simulink model "finalmodel1"  (R2024b)
settings: Solver=FixedStepDiscrete  StartTime=0.0  StopTime=110  FixedStep=SampleTime  MaxStep=1e-3  RelTol=1e-4  AbsTol=1e-3
InitFcn:
  | Ts=50e-6; SampleTime=50e-6; PSSMODEL=1;
  | MB=[1   0.2 30   1.25 40    12 160];
  | 
  | k=[8.3222    2.6014   19.0811    1.9818    3.6841   19.1783  240.6785    2.5684    4.3666   58.7391 7.6960   47.7975    8.7139  296.2463    2.7543    6.5051   47.7755    0.4780   35.4950   18.1866 94.2186]
  | k1=k(1);
  | k2=k(2);
  | k3=k(3);
  | k4=k(4);
  | k5=k(5);
  | k6=k(6);
  | k7=k(7);
  | k8=k(8);
  | k9=k(9);
  | k10=k(10);
  | k11=k(11);
  | k12=k(12);
  | k13=k(13);
  | k14=k(14);
  | k15=k(15);
  | k16=k(16);
  | k17=k(17);
  | k18=k(18);
  | k19=k(19);
  | k20=k(20);
  | k21=k(21);
undefined symbols (not defined in the file or in its folder): dEgdT, DiscIntNeverNeededParam, EgRef, gcbh, Rsh_array5pc, sigbuilder_block, sps_rtmsupport, Tref_K, VT_ref
libraries: spsThreePhaseVIMeasurementLib x14, spsLoadFlowBusLib x9, spsThreePhasePISectionLineLib x6, spsSeriesRLCBranchLib x5, spsThreePhaseTransformerTwoWindingsLib x4, slpidlib x4, spsThreePhaseParallelRLCLoadLib x4, spsThreePhaseSeriesRLCBranchLib x3, spsAlphaBetaZerotodq0Lib x2, spsSynchronousMachinepuStandardLib x2, spsExcitationSystemLib x2, spsMultiBandPowerSystemStabilizerLib x2
(part 1 of 9)
settings Model: Creator=jp536285  LastModifiedBy=Raju
settings SolverCC: AutoScaleAbsTol=off  InitialStep=1e-5  ZeroCrossControl=DisableAll  AlgebraicLoopSolver=TrustRegion  AutoInsertRateTranBlk=on
settings DataIOCC: MaxDataPoints=100000
settings OptimizationCC: LifeSpan=inf
settings DebuggingCC: UnderspecifiedInitializationDetection=Classic  MergeDetectMultiDrivingBlocksExec=none  MultiTaskRateTransMsg=warning  IntegerOverflowMsg=none  StateNameClashWarn=warning  SFUnexpectedBacktrackingDiag=warning  SFNoUnconditionalDefaultTransitionDiag=warning  ArithmeticOperatorsInVariantConditions=warning
settings HardwareCC: ProdBitPerPointer=32  ProdBitPerSizeT=32  ProdBitPerPtrDiffT=32  ProdLargestAtomicFloat=None  ProdIntDivRoundTo=Undefined  ProdEndianess=Unspecified  ProdWordSize=32  ProdHWDeviceType=32-bit Generic
settings ModelReferenceCC: EnableRefExpFcnMdlSchedulingChecks=on  PropagateSignalLabelsOutOfModel=off
settings SFSimCC: SimUseLocalCustomCode=off  CustomCodeUndefinedFunction=UseInterfaceOnly
settings RTWCC: RTWUseLocalCustomCode=off  GPUComputeCapability=3.5
settings CodeAppCC: StateflowObjectComments=on
settings GRTTargetCC: TargetLangStandard=C89/C90 (ANSI)
settings ConfigComp: CovMetricSettings=dw  CovSaveCumulativeToWorkspaceVar=on  CovSaveSingleToWorkspaceVar=on  CovExternalEMLEnable=off
settings SimscapeCC: SimscapeNormalizeSystem=off

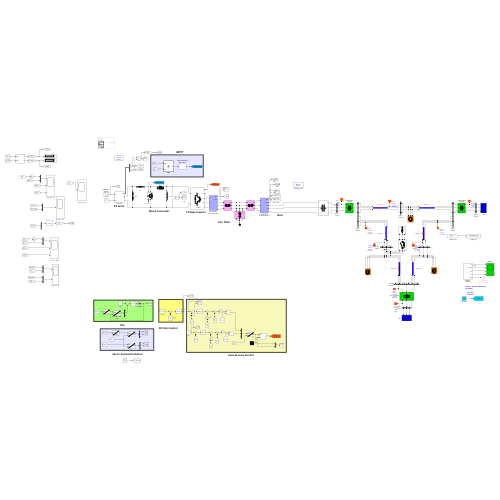
[thumbnail: Simulink's stored preview of the top-level diagram]
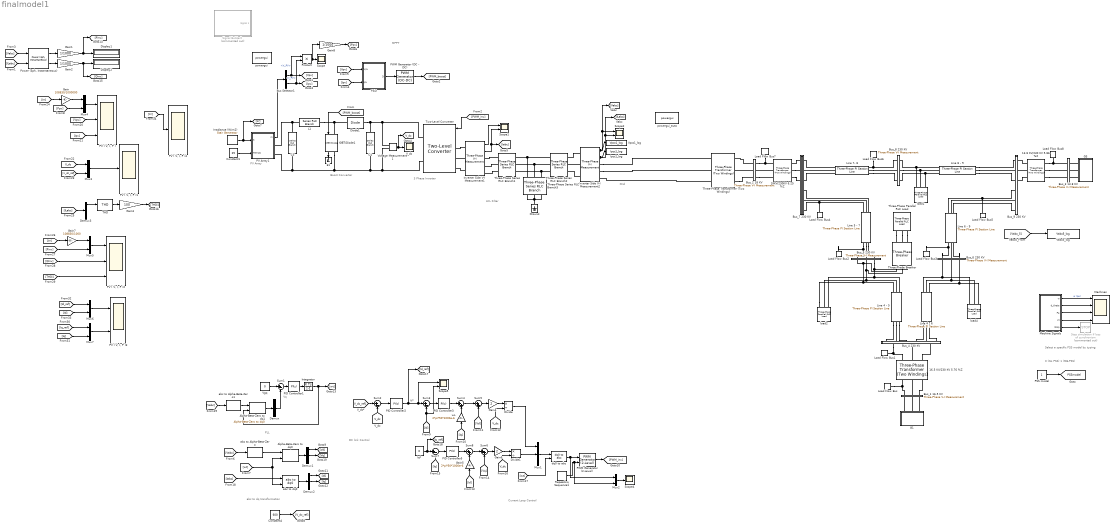
== system finalmodel1 ==
  note: Select a specific PSS model
      | by typing:
  note: 0  (No PSS)
      | 1  (MB-PSS)
  note: DC link Control
  note: Grid
  note: PLL
  note: abc to dq transformation
  note: 3 Phase Inverter
  note: LCL Filter
  note: Boost Converter
  note: PV Array
  note: Id*
  note: Current Loop Control
  note: MPPT
  note: Vq
  " Line 4 - 6" : spsThreePhasePISectionLineLib/Three-Phase PI Section Line  LConnTagsString=a|b|c  RConnTagsString=A|B|C  Length=100  Frequency=60  Resistances=[ 0.08993 0.224825]  Inductances="[ 1.29e-3  3.22e-3]"  Capacitances="[ 9.5e-9  6.5e-9 ]"  mask(Three-Phase PI Section Line){}
      mask Display:
      | % This is a new mask on top of the base mask.
      | % Use "View base mask" link below to see the base mask.
      | patch([0.0 0.0 1 1 0.0 0.0 ],[0.4 0.7 0.7 0.4 0.4 0.7],[0 0 1]);
      | patch([0.4 0.4 0.42 0.42],[0.4 0.75 0.75 0.4],[1 0 0]);
      | patch([0.38 0.38 0.57 0.57],[0.7 0.75 0.75 0.7],[1 0 0]);
      | patch([0.53 0.53 0.55 0.55],[0.4 0.75 0.75 0.4],[1 0 0]);
  " Line 6 - 9" : spsThreePhasePISectionLineLib/Three-Phase PI Section Line  LConnTagsString=a|b|c  RConnTagsString=A|B|C  Length=100  Frequency=60  Resistances=[ 0.20631 0.5157]  Inductances="[ 2.38e-3  6.09e-3]"  Capacitances=[17.95e-9 10.55e-9]  mask(Three-Phase PI Section Line){}
      mask Display:
      | % This is a new mask on top of the base mask.
      | % Use "View base mask" link below to see the base mask.
      | patch([0.0 0.0 1 1 0.0 0.0 ],[0.4 0.7 0.7 0.4 0.4 0.7],[0 0 1]);
      | patch([0.4 0.4 0.42 0.42],[0.4 0.75 0.75 0.4],[1 0 0]);
      | patch([0.38 0.38 0.57 0.57],[0.7 0.75 0.75 0.7],[1 0 0]);
      | patch([0.53 0.53 0.55 0.55],[0.4 0.75 0.75 0.4],[1 0 0]);
  13.8 KV/230 KV 5.86 %Z : spsThreePhaseTransformerTwoWindingsLib/Three-Phase Transformer (Two Windings)  Winding1Connection=Yg  Winding2Connection=Yg  CoreType=Three single-phase transformers  SetSaturation=off  Hysteresis=off  DataFile='hysteresis'  SetInitialFlux=off  Measurements=None  UNITS=pu  NominalPower=[ 100e6 , 60 ]  Winding1=[ 13.8e3 , 1e-6 , 0 ]  Winding2=[ 230e3 , 1e-6, 0.0586 ]  Rm=500  Lm=500  L0=0.5  Saturation=[ 0,0 ; 0.0024,1.2 ; 1.0,1.52 ]  InitialFluxes=[ 0.8 , -0.8 , 0.7 ]  BreakLoop=off  DiscreteSolver=Trapezoidal iterative  DataType=off  TransfoNumber=1
  "16.5 KV/230 KV 5.76 %Z     " : spsThreePhaseTransformerTwoWindingsLib/Three-Phase Transformer (Two Windings)  Winding1Connection=Yg  Winding2Connection=Yg  CoreType=Three single-phase transformers  SetSaturation=off  Hysteresis=off  DataFile='hysteresis'  SetInitialFlux=off  Measurements=None  UNITS=pu  NominalPower=[ 100e6 , 60 ]  Winding1=[ 16.5e3 , 1e-6, 0 ]  Winding2=[ 230e3 ,1e-6, 0.0576 ]  Rm=500  Lm=500  L0=0.5  Saturation=[ 0,0 ; 0.0024,1.2 ; 1.0,1.52 ]  InitialFluxes=[ 0.8 , -0.8 , 0.7 ]  BreakLoop=off  DiscreteSolver=Trapezoidal iterative  DataType=off  TransfoNumber=1
  18KV/230KV 6.25 %Z : spsThreePhaseTransformerTwoWindingsLib/Three-Phase Transformer (Two Windings)  Winding1Connection=Yg  Winding2Connection=Yg  CoreType=Three single-phase transformers  SetSaturation=off  Hysteresis=off  DataFile='hysteresis'  SetInitialFlux=off  Measurements=None  UNITS=pu  NominalPower=[ 100e6 , 60 ]  Winding1=[ 18e3 , 1e-6 , 0]  Winding2=[ 230e3 , 1e-6, 0.0625 ]  Rm=500  Lm=500  L0=0.5  Saturation=[ 0,0 ; 0.0024,1.2 ; 1.0,1.52 ]  InitialFluxes=[ 0.8 , -0.8 , 0.7 ]  BreakLoop=off  DiscreteSolver=Trapezoidal iterative  DataType=off  TransfoNumber=1
  Alpha-Beta-Zero to dq0 : spsAlphaBetaZerotodq0Lib/Alpha-Beta-Zero to dq0  Alignment=90 degrees behind phase A axis
  Alpha-Beta-Zero to dq1 : spsAlphaBetaZerotodq0Lib/Alpha-Beta-Zero to dq0  Alignment=90 degrees behind phase A axis
  Bus Selector1 : BusSelector  OutputSignals=V_PV,I_PV
  Bus_1 16.5 KV : spsThreePhaseVIMeasurementLib/Three-Phase V-I Measurement  VoltageMeasurement=phase-to-ground  SetLabelV=on  LabelV=Vabc_1  Vpu=on  VpuLL=off  CurrentMeasurement=yes  SetLabelI=on  LabelI=Iabc_1  Ipu=on  Pbase=100e6  Vbase=16.5e3  OutputType=Complex  PhasorSimulation=off  PSBequivalent=0
  Bus_2 18 KV : spsThreePhaseVIMeasurementLib/Three-Phase V-I Measurement  VoltageMeasurement=phase-to-ground  SetLabelV=on  LabelV=Vabc_2  Vpu=on  VpuLL=off  CurrentMeasurement=yes  SetLabelI=on  LabelI=Iabc_2  Ipu=on  Pbase=100e6  Vbase=18e3  OutputType=Complex  PhasorSimulation=off  PSBequivalent=0
  Bus_3 13.8 KV : spsThreePhaseVIMeasurementLib/Three-Phase V-I Measurement  VoltageMeasurement=phase-to-ground  SetLabelV=on  LabelV=Vabc_3  Vpu=on  VpuLL=off  CurrentMeasurement=yes  SetLabelI=on  LabelI=Iabc_3  Ipu=on  Pbase=100e6  Vbase=13.8e3  OutputType=Complex  PhasorSimulation=off  PSBequivalent=0
  Bus_4 230 KV : Subsystem
  Bus_5 230 KV : spsThreePhaseVIMeasurementLib/Three-Phase V-I Measurement  VoltageMeasurement=phase-to-ground  SetLabelV=on  LabelV=Vabc_5  Vpu=on  VpuLL=off  CurrentMeasurement=yes  SetLabelI=on  LabelI=Iabc_5  Ipu=on  Pbase=100e6  Vbase=230e3  OutputType=Complex  PhasorSimulation=off  PSBequivalent=0
  Bus_6 230 KV : spsThreePhaseVIMeasurementLib/Three-Phase V-I Measurement  VoltageMeasurement=phase-to-phase  SetLabelV=on  LabelV=Vabc_6  Vpu=off  VpuLL=on  CurrentMeasurement=yes  SetLabelI=on  LabelI=Iabc_6  Ipu=on  Pbase=100e6  Vbase=230e3  OutputType=Complex  PhasorSimulation=off  PSBequivalent=0
  Bus_7 230 KV : Subsystem
  Bus_8 230 KV : spsThreePhaseVIMeasurementLib/Three-Phase V-I Measurement  VoltageMeasurement=phase-to-phase  SetLabelV=on  LabelV=Vabc_8  Vpu=off  VpuLL=on  CurrentMeasurement=yes  SetLabelI=on  LabelI=Iabc_8  Ipu=on  Pbase=100e6  Vbase=230e3  OutputType=Complex  PhasorSimulation=off  PSBequivalent=0
  Bus_9 230 KV : Subsystem
  C3 : spsSeriesRLCBranchLib/Series RLC Branch  LConnTagsString=__new0  RConnTagsString=__new0  BranchType=RC  Resistance=1e-3  Inductance=1e-3  SetiL0=off  InitialCurrent=0  Capacitance=1000e-6  Setx0=off  InitialVoltage=0  Measurements=None
  C4 : spsSeriesRLCBranchLib/Series RLC Branch  LConnTagsString=__new0  RConnTagsString=__new0  BranchType=C  Resistance=1  Inductance=1e-3  SetiL0=off  InitialCurrent=0  Capacitance=3227e-6  Setx0=off  InitialVoltage=3227e-6  Measurements=None
  Constant1 : Constant  Value=25  SampleTime=SampleTime
  Constant4 : Constant  Value=600  SampleTime=SampleTime
  Demux{,1..3} (4 alike) : Demux  Outputs=3
  Diode1 : spsDiodeLib/Diode  Ron=0.001  Lon=0  Vf=0.8  IC=0  UseSnubber=off  Rs=500  Cs=250e-9  Measurements=off
  Display1 : Display
      settings: SampleTime=SampleTime
  Display2 : Display
      settings: SampleTime=SampleTime
  Divide : Product  Inputs=*/  SampleTime=SampleTime
  Divide1 : Product  Inputs=*/  SampleTime=SampleTime
  E1 : Terminator
  G1 : Subsystem
  G3 : Subsystem
  Gain : Gain  Gain=108830/1000000  SampleTime=SampleTime
  Gain1 : Gain  Gain=1/1000  SampleTime=SampleTime
  Gain2 : Gain  Gain=1/1000  SampleTime=SampleTime
  Gain3 : Gain  Gain=100  SampleTime=SampleTime
  Gain4 : Gain  Gain=2  SampleTime=SampleTime
  Gain5 : Gain  Gain=2*pi*50*1000e-6  SampleTime=SampleTime
  Gain6 : Gain  Gain=2  SampleTime=SampleTime
  Gain7 : Gain  Gain=108830/1000  SampleTime=SampleTime
  Gain8 : Gain  Gain=1/1000  SampleTime=SampleTime
  "Ground " : spsGroundLib/Ground  LConnTagsString=a
  IGBT/Diode1 : spsIGBTDiodeLib/IGBT//Diode  Ron=1e-3  Rs=1e5  Cs=inf  Measurements=on
  Integrator : DiscreteIntegrator  SampleTime=SampleTime  ICPrevOutput=DiscIntNeverNeededParam  ICPrevScaledInput=DiscIntNeverNeededParam
  Inverter Side V-I Measurement1 : spsThreePhaseVIMeasurementLib/Three-Phase V-I Measurement  VoltageMeasurement=phase-to-phase  SetLabelV=off  LabelV=Vabc  Vpu=off  VpuLL=off  CurrentMeasurement=yes  SetLabelI=off  LabelI=Iabc  Ipu=off  Pbase=100e6  Vbase=500e3  OutputType=Complex  PhasorSimulation=off  PSBequivalent=0
  Inverter Side V-I Measurement2 : spsThreePhaseVIMeasurementLib/Three-Phase V-I Measurement  VoltageMeasurement=phase-to-ground  SetLabelV=off  LabelV=Vabc  Vpu=off  VpuLL=off  CurrentMeasurement=yes  SetLabelI=off  LabelI=Iabc  Ipu=off  Pbase=100e6  Vbase=500e3  OutputType=Complex  PhasorSimulation=off  PSBequivalent=0
  Ipcc1_log : ToWorkspace  VariableName=Ipcc1_log  SaveFormat=Timeseries  SampleTime=-1
  Iq* : Constant  Value=0  SampleTime=SampleTime
  Irradiance (W/m2) : spsStairGeneratorLib/Stair Generator  t=[0, 0.1 , 0.2 , 0.3, 0.4]  e=[1, 1, 0.4, 1, 1]*1000  Ts=SampleTime
      link override Model/Digital Clock: SampleTime=SampleTime
      link override Model/Look-Up Table: SampleTime=SampleTime
      link override Out: SampleTime=SampleTime
  L1 : spsSeriesRLCBranchLib/Series RLC Branch  LConnTagsString=__new0  RConnTagsString=__new0  BranchType=L  Resistance=1  Inductance=1.45e-3  SetiL0=off  InitialCurrent=250  Capacitance=1e-6  Setx0=off  InitialVoltage=0  Measurements=None
  "Line 4 - 5 " : spsThreePhasePISectionLineLib/Three-Phase PI Section Line  LConnTagsString=a|b|c  RConnTagsString=A|B|C  Length=100  Frequency=60  Resistances=[ 0.0529 0.13225]  Inductances="[ 1.192e-3  2.38e-3]"  Capacitances="[ 9.5e-9  6.5e-9 ]"  mask(Three-Phase PI Section Line){}
      mask Display:
      | % This is a new mask on top of the base mask.
      | % Use "View base mask" link below to see the base mask.
      | patch([0.0 0.0 1 1 0.0 0.0 ],[0.4 0.7 0.7 0.4 0.4 0.7],[0 0 1]);
      | patch([0.4 0.4 0.42 0.42],[0.4 0.75 0.75 0.4],[1 0 0]);
      | patch([0.38 0.38 0.57 0.57],[0.7 0.75 0.75 0.7],[1 0 0]);
      | patch([0.53 0.53 0.55 0.55],[0.4 0.75 0.75 0.4],[1 0 0]);
  "Line 5 - 7 " : spsThreePhasePISectionLineLib/Three-Phase PI Section Line  LConnTagsString=a|b|c  RConnTagsString=A|B|C  Length=100  Frequency=60  Resistances=[ 0.16928 0.4232]  Inductances="[ 2.259e-3  5.64e-3]"  Capacitances=[15.34e-9 9.025e-9]  mask(Three-Phase PI Section Line){}
      mask Display:
      | % This is a new mask on top of the base mask.
      | % Use "View base mask" link below to see the base mask.
      | patch([0.0 0.0 1 1 0.0 0.0 ],[0.4 0.7 0.7 0.4 0.4 0.7],[0 0 1]);
      | patch([0.4 0.4 0.42 0.42],[0.4 0.75 0.75 0.4],[1 0 0]);
      | patch([0.38 0.38 0.57 0.57],[0.7 0.75 0.75 0.7],[1 0 0]);
      | patch([0.53 0.53 0.55 0.55],[0.4 0.75 0.75 0.4],[1 0 0]);
  Line 7- 8 : spsThreePhasePISectionLineLib/Three-Phase PI Section Line  LConnTagsString=a|b|c  RConnTagsString=A|B|C  Length=100  Frequency=60  Resistances=[0.044965 0.11241]  Inductances="[ 1.01e-3  2.02e-3]"  Capacitances="[ 12.5e-9  6.5e-9 ]"  mask(Three-Phase PI Section Line){}
      mask Display:
      | % This is a new mask on top of the base mask.
      | % Use "View base mask" link below to see the base mask.
      | patch([0.0 0.0 1 1 0.0 0.0 ],[0.4 0.7 0.7 0.4 0.4 0.7],[0 0 1]);
      | patch([0.4 0.4 0.42 0.42],[0.4 0.75 0.75 0.4],[1 0 0]);
      | patch([0.38 0.38 0.57 0.57],[0.7 0.75 0.75 0.7],[1 0 0]);
      | patch([0.53 0.53 0.55 0.55],[0.4 0.75 0.75 0.4],[1 0 0]);
  Line 8 - 9 : spsThreePhasePISectionLineLib/Three-Phase PI Section Line  LConnTagsString=a|b|c  RConnTagsString=A|B|C  Length=100  Frequency=60  Resistances=[ 0.062951 0.15737]  Inductances="[ 1.414e-3  3.53e-3]"  Capacitances=[10.47e-9 6.15e-9]  mask(Three-Phase PI Section Line){}
      mask Display:
      | % This is a new mask on top of the base mask.
      | % Use "View base mask" link below to see the base mask.
      | patch([0.0 0.0 1 1 0.0 0.0 ],[0.4 0.7 0.7 0.4 0.4 0.7],[0 0 1]);
      | patch([0.4 0.4 0.42 0.42],[0.4 0.75 0.75 0.4],[1 0 0]);
      | patch([0.38 0.38 0.57 0.57],[0.7 0.75 0.75 0.7],[1 0 0]);
      | patch([0.53 0.53 0.55 0.55],[0.4 0.75 0.75 0.4],[1 0 0]);
  Load Flow Bus : spsLoadFlowBusLib/Load Flow Bus  LConnTagsString=a  Phases=single  Connectors=on one side  ID=BUS_1  Vbase=16.5e3  Vref=1.04  Vangle=0  VLF=1.04  VLFb=1  VLFc=1  angleLF=0  angleLFb=0  angleLFc=0
      settings: AttributesFormatString=%<ID>\n%<Vbase>V\n%<VLF>pu\n%<angleLF>deg.
  Load Flow Bus1 : spsLoadFlowBusLib/Load Flow Bus  LConnTagsString=a  Phases=single  Connectors=on one side  ID=BUS_4  Vbase=230e3  Vref=1  Vangle=0  VLF=1.029  VLFb=1  VLFc=1  angleLF=-7.275  angleLFb=0  angleLFc=0
      settings: AttributesFormatString=%<ID>\n%<Vbase>V\n%<VLF>pu\n%<angleLF>deg.
  Load Flow Bus2 : spsLoadFlowBusLib/Load Flow Bus  LConnTagsString=a  Phases=single  Connectors=on one side  ID=BUS_5  Vbase=230e3  Vref=1  Vangle=0  VLF=1.002  VLFb=1  VLFc=1  angleLF=-13.97  angleLFb=0  angleLFc=0
      settings: AttributesFormatString=%<ID>\n%<Vbase>V\n%<VLF>pu\n%<angleLF>deg.
  Load Flow Bus3 : spsLoadFlowBusLib/Load Flow Bus  LConnTagsString=a  Phases=single  Connectors=on one side  ID=BUS_6  Vbase=230e3  Vref=1  Vangle=0  VLF=1.017  VLFb=1  VLFc=1  angleLF=-11.82  angleLFb=0  angleLFc=0
      settings: AttributesFormatString=%<ID>\n%<Vbase>V\n%<VLF>pu\n%<angleLF>deg.
  Load Flow Bus4 : spsLoadFlowBusLib/Load Flow Bus  LConnTagsString=a  Phases=single  Connectors=on one side  ID=BUS_7  Vbase=230e3  Vref=1  Vangle=0  VLF=1.025  VLFb=1  VLFc=1  angleLF=-15.86  angleLFb=0  angleLFc=0
      settings: AttributesFormatString=%<ID>\n%<Vbase>V\n%<VLF>pu\n%<angleLF>deg.
  Load Flow Bus5 : spsLoadFlowBusLib/Load Flow Bus  LConnTagsString=a  Phases=single  Connectors=on one side  ID=BUS_9  Vbase=230e3  Vref=1  Vangle=0  VLF=1.031  VLFb=1  VLFc=1  angleLF=-11.92  angleLFb=0  angleLFc=0
      settings: AttributesFormatString=%<ID>\n%<Vbase>V\n%<VLF>pu\n%<angleLF>deg.
  Load Flow Bus6 : spsLoadFlowBusLib/Load Flow Bus  LConnTagsString=a  Phases=single  Connectors=on one side  ID=BUS_8  Vbase=230e3  Vref=1  Vangle=0  VLF=1.017  VLFb=1  VLFc=1  angleLF=-16.48  angleLFb=0  angleLFc=0
      settings: AttributesFormatString=%<ID>\n%<Vbase>V\n%<VLF>pu\n%<angleLF>deg.
  Load Flow Bus7 : spsLoadFlowBusLib/Load Flow Bus  LConnTagsString=a  Phases=single  Connectors=on one side  ID=BUS_2  Vbase=18e3  Vref=1.025  Vangle=0  VLF=1.025  VLFb=1  VLFc=1  angleLF=-15.88  angleLFb=0  angleLFc=0
      settings: AttributesFormatString=%<ID>\n%<Vbase>V\n%<VLF>pu\n%<angleLF>deg.
  Load Flow Bus8 : spsLoadFlowBusLib/Load Flow Bus  LConnTagsString=a  Phases=single  Connectors=on one side  ID=BUS_3  Vbase=13.8e3  Vref=1.025  Vangle=0  VLF=1.025  VLFb=1  VLFc=1  angleLF=-9.229  angleLFb=0  angleLFc=0
      settings: AttributesFormatString=%<ID>\n%<Vbase>V\n%<VLF>pu\n%<angleLF>deg.
  Machine Signals : Subsystem
  Machines : Scope  NumInputPorts=4
  Mux1 : Mux  Inputs=3
  Mux{2..7} (6 alike) : Mux  Inputs=2
  P&O : MATLAB Function  TreatAsAtomicUnit=on
  PID Controller1 : slpidlib/PID Controller  Controller=PI  Form=Parallel  TimeDomain=Discrete-time  UseExternalTs=off  SampleTime=SampleTime  IntegratorMethod=Forward Euler  FilterMethod=Forward Euler  ControllerParametersSource=internal  P=10  I=50000  UseKiTs=off  D=0  UseExternalDerivativeSource=off  N=100  UseFilter=on  TunerSelectOption=Transfer Function Based (PID Tuner App)  InitialConditionSource=internal  InitialConditionForIntegrator=0  InitialConditionForFilter=0  DifferentiatorICPrevScaledInput=0  ExternalReset=none  TrackingMode=off  Kt=1  LimitOutput=off  SatLimitsSource=internal  UpperSaturationLimit=inf  LowerSaturationLimit=-inf  LinearizeAsGain=on  AntiWindupMode=none  Kb=1  LimitIntegrator=off  UpperIntegratorSaturationLimit=inf  LowerIntegratorSaturationLimit=-inf  POutMin=[]  POutMax=[]  IOutMin=[]  IOutMax=[]  DOutMin=[]  DOutMax=[]  NOutMin=[]  NOutMax=[]  SumOutMin=[]  SumOutMax=[]  SaturationOutMin=[]  SaturationOutMax=[]  PParamMin=[]  PParamMax=[]  IParamMin=[]  IParamMax=[]  DParamMin=[]  DParamMax=[]  NParamMin=[]  NParamMax=[]  KbParamMin=[]  KbParamMax=[]  KtParamMin=[]  KtParamMax=[]  KbOutMin=[]  KbOutMax=[]  KtOutMin=[]  KtOutMax=[]  IntegratorOutMin=[]  IntegratorOutMax=[]  FilterOutMin=[]  FilterOutMax=[]  SumI1OutMin=[]  SumI1OutMax=[]  SumI2OutMin=[]  SumI2OutMax=[]  SumI3OutMin=[]  SumI3OutMax=[]  SumI4OutMin=[]  SumI4OutMax=[]  SumDOutMin=[]  SumDOutMax=[]  DifferentiatorOutMin=[]  DifferentiatorOutMax=[]  FilterDiffOutCoefMin=[]  FilterDiffOutCoefMax=[]  ReciprocalOutMin=[]  ReciprocalOutMax=[]  SumDenOutMin=[]  SumDenOutMax=[]  SumNumOutMin=[]  SumNumOutMax=[]  DivideOutMin=[]  DivideOutMax=[]  UdiffTsProdOutMin=[]  UdiffTsProdOutMax=[]  NTsProdOutMin=[]  NTsProdOutMax=[]  UintegralTsProdOutMin=[]  UintegralTsProdOutMax=[]  UngainTsProdOutMin=[]  UngainTsProdOutMax=[]  ClampingZeroOutDataTypeStr=Inherit: Inherit via back propagation  ClampingZeroOutMin=[]  ClampingZeroOutMax=[]  FilterDenConstantOutDataTypeStr=Inherit: Inherit via back propagation  FilterDenConstantOutMin=[]  FilterDenConstantOutMax=[]  PCopyOutDataTypeStr=Inherit: Inherit via back propagation  PCopyOutMin=[]  PCopyOutMax=[]  NCopyOutDataTypeStr=Inherit: Inherit via back propagation  NCopyOutMin=[]  NCopyOutMax=[]  IntegratorContinuousStateAttributes=''  IntegratorStateMustResolveToSignalObject=off  IntegratorRTWStateStorageClass=Auto  FilterContinuousStateAttributes=''  FilterStateMustResolveToSignalObject=off  FilterRTWStateStorageClass=Auto  ParallelPVariant=InternalParameters  IdealPVariant=Disabled  IVariant=InternalParameters  DVariant=Disabled  IntegratorVariant=Discrete  SatVariant=Disabled  AWVariant=Passthrough  PCopyVariant=Disabled  TRVariant=Disabled  FdbkBlocksVariant=Forward  IdealPFdbkVariant=Disabled  SatFdbkVariant=Disabled  DerivativeFilterVariant=Disabled  NVariant=Disabled  NCopyVariant=Disabled_SignalSpec  FilterICVariant=Disabled  IntegratorICVariant=InternalICs  ExternalResetVariant=Disabled  TRSumVariant=Passthrough  SumFdbkVariant=Disabled  SumVariant=Sum_PI  TsampFilterVariant=InternalTs  TsampNgainVariant=Passthrough  TsampIntegralVariant=Disabled_SignalSpec  ExternalSaturationOutDataTypeStr=Inherit: Same as second input  DerivativeSourceVariant=Disabled  PreIntVariant=InternalPreInt
  PID Controller2 : slpidlib/PID Controller  Controller=PI  Form=Parallel  TimeDomain=Discrete-time  UseExternalTs=off  SampleTime=SampleTime  IntegratorMethod=Forward Euler  FilterMethod=Forward Euler  ControllerParametersSource=internal  P=0.25  I=300  UseKiTs=off  D=0  UseExternalDerivativeSource=off  N=100  UseFilter=on  TunerSelectOption=Transfer Function Based (PID Tuner App)  InitialConditionSource=internal  InitialConditionForIntegrator=0  InitialConditionForFilter=0  DifferentiatorICPrevScaledInput=0  ExternalReset=none  TrackingMode=off  Kt=1  LimitOutput=off  SatLimitsSource=internal  UpperSaturationLimit=inf  LowerSaturationLimit=-inf  LinearizeAsGain=on  AntiWindupMode=none  Kb=1  LimitIntegrator=off  UpperIntegratorSaturationLimit=inf  LowerIntegratorSaturationLimit=-inf  POutMin=[]  POutMax=[]  IOutMin=[]  IOutMax=[]  DOutMin=[]  DOutMax=[]  NOutMin=[]  NOutMax=[]  SumOutMin=[]  SumOutMax=[]  SaturationOutMin=[]  SaturationOutMax=[]  PParamMin=[]  PParamMax=[]  IParamMin=[]  IParamMax=[]  DParamMin=[]  DParamMax=[]  NParamMin=[]  NParamMax=[]  KbParamMin=[]  KbParamMax=[]  KtParamMin=[]  KtParamMax=[]  KbOutMin=[]  KbOutMax=[]  KtOutMin=[]  KtOutMax=[]  IntegratorOutMin=[]  IntegratorOutMax=[]  FilterOutMin=[]  FilterOutMax=[]  SumI1OutMin=[]  SumI1OutMax=[]  SumI2OutMin=[]  SumI2OutMax=[]  SumI3OutMin=[]  SumI3OutMax=[]  SumI4OutMin=[]  SumI4OutMax=[]  SumDOutMin=[]  SumDOutMax=[]  DifferentiatorOutMin=[]  DifferentiatorOutMax=[]  FilterDiffOutCoefMin=[]  FilterDiffOutCoefMax=[]  ReciprocalOutMin=[]  ReciprocalOutMax=[]  SumDenOutMin=[]  SumDenOutMax=[]  SumNumOutMin=[]  SumNumOutMax=[]  DivideOutMin=[]  DivideOutMax=[]  UdiffTsProdOutMin=[]  UdiffTsProdOutMax=[]  NTsProdOutMin=[]  NTsProdOutMax=[]  UintegralTsProdOutMin=[]  UintegralTsProdOutMax=[]  UngainTsProdOutMin=[]  UngainTsProdOutMax=[]  ClampingZeroOutDataTypeStr=Inherit: Inherit via back propagation  ClampingZeroOutMin=[]  ClampingZeroOutMax=[]  FilterDenConstantOutDataTypeStr=Inherit: Inherit via back propagation  FilterDenConstantOutMin=[]  FilterDenConstantOutMax=[]  PCopyOutDataTypeStr=Inherit: Inherit via back propagation  PCopyOutMin=[]  PCopyOutMax=[]  NCopyOutDataTypeStr=Inherit: Inherit via back propagation  NCopyOutMin=[]  NCopyOutMax=[]  IntegratorContinuousStateAttributes=''  IntegratorStateMustResolveToSignalObject=off  IntegratorRTWStateStorageClass=Auto  FilterContinuousStateAttributes=''  FilterStateMustResolveToSignalObject=off  FilterRTWStateStorageClass=Auto  ParallelPVariant=InternalParameters  IdealPVariant=Disabled  IVariant=InternalParameters  DVariant=Disabled  IntegratorVariant=Discrete  SatVariant=Disabled  AWVariant=Passthrough  PCopyVariant=Disabled  TRVariant=Disabled  FdbkBlocksVariant=Forward  IdealPFdbkVariant=Disabled  SatFdbkVariant=Disabled  DerivativeFilterVariant=Disabled  NVariant=Disabled  NCopyVariant=Disabled_SignalSpec  FilterICVariant=Disabled  IntegratorICVariant=InternalICs  ExternalResetVariant=Disabled  TRSumVariant=Passthrough  SumFdbkVariant=Disabled  SumVariant=Sum_PI  TsampFilterVariant=InternalTs  TsampNgainVariant=Passthrough  TsampIntegralVariant=Disabled_SignalSpec  ExternalSaturationOutDataTypeStr=Inherit: Same as second input  DerivativeSourceVariant=Disabled  PreIntVariant=InternalPreInt
  PID Controller3 : slpidlib/PID Controller  Controller=PI  Form=Parallel  TimeDomain=Discrete-time  UseExternalTs=off  SampleTime=SampleTime  IntegratorMethod=Forward Euler  FilterMethod=Forward Euler  ControllerParametersSource=internal  P=10  I=20  UseKiTs=off  D=0  UseExternalDerivativeSource=off  N=100  UseFilter=on  TunerSelectOption=Transfer Function Based (PID Tuner App)  InitialConditionSource=internal  InitialConditionForIntegrator=0  InitialConditionForFilter=0  DifferentiatorICPrevScaledInput=0  ExternalReset=none  TrackingMode=off  Kt=1  LimitOutput=off  SatLimitsSource=internal  UpperSaturationLimit=inf  LowerSaturationLimit=-inf  LinearizeAsGain=on  AntiWindupMode=none  Kb=1  LimitIntegrator=off  UpperIntegratorSaturationLimit=inf  LowerIntegratorSaturationLimit=-inf  POutMin=[]  POutMax=[]  IOutMin=[]  IOutMax=[]  DOutMin=[]  DOutMax=[]  NOutMin=[]  NOutMax=[]  SumOutMin=[]  SumOutMax=[]  SaturationOutMin=[]  SaturationOutMax=[]  PParamMin=[]  PParamMax=[]  IParamMin=[]  IParamMax=[]  DParamMin=[]  DParamMax=[]  NParamMin=[]  NParamMax=[]  KbParamMin=[]  KbParamMax=[]  KtParamMin=[]  KtParamMax=[]  KbOutMin=[]  KbOutMax=[]  KtOutMin=[]  KtOutMax=[]  IntegratorOutMin=[]  IntegratorOutMax=[]  FilterOutMin=[]  FilterOutMax=[]  SumI1OutMin=[]  SumI1OutMax=[]  SumI2OutMin=[]  SumI2OutMax=[]  SumI3OutMin=[]  SumI3OutMax=[]  SumI4OutMin=[]  SumI4OutMax=[]  SumDOutMin=[]  SumDOutMax=[]  DifferentiatorOutMin=[]  DifferentiatorOutMax=[]  FilterDiffOutCoefMin=[]  FilterDiffOutCoefMax=[]  ReciprocalOutMin=[]  ReciprocalOutMax=[]  SumDenOutMin=[]  SumDenOutMax=[]  SumNumOutMin=[]  SumNumOutMax=[]  DivideOutMin=[]  DivideOutMax=[]  UdiffTsProdOutMin=[]  UdiffTsProdOutMax=[]  NTsProdOutMin=[]  NTsProdOutMax=[]  UintegralTsProdOutMin=[]  UintegralTsProdOutMax=[]  UngainTsProdOutMin=[]  UngainTsProdOutMax=[]  ClampingZeroOutDataTypeStr=Inherit: Inherit via back propagation  ClampingZeroOutMin=[]  ClampingZeroOutMax=[]  FilterDenConstantOutDataTypeStr=Inherit: Inherit via back propagation  FilterDenConstantOutMin=[]  FilterDenConstantOutMax=[]  PCopyOutDataTypeStr=Inherit: Inherit via back propagation  PCopyOutMin=[]  PCopyOutMax=[]  NCopyOutDataTypeStr=Inherit: Inherit via back propagation  NCopyOutMin=[]  NCopyOutMax=[]  IntegratorContinuousStateAttributes=''  IntegratorStateMustResolveToSignalObject=off  IntegratorRTWStateStorageClass=Auto  FilterContinuousStateAttributes=''  FilterStateMustResolveToSignalObject=off  FilterRTWStateStorageClass=Auto  ParallelPVariant=InternalParameters  IdealPVariant=Disabled  IVariant=InternalParameters  DVariant=Disabled  IntegratorVariant=Discrete  SatVariant=Disabled  AWVariant=Passthrough  PCopyVariant=Disabled  TRVariant=Disabled  FdbkBlocksVariant=Forward  IdealPFdbkVariant=Disabled  SatFdbkVariant=Disabled  DerivativeFilterVariant=Disabled  NVariant=Disabled  NCopyVariant=Disabled_SignalSpec  FilterICVariant=Disabled  IntegratorICVariant=InternalICs  ExternalResetVariant=Disabled  TRSumVariant=Passthrough  SumFdbkVariant=Disabled  SumVariant=Sum_PI  TsampFilterVariant=InternalTs  TsampNgainVariant=Passthrough  TsampIntegralVariant=Disabled_SignalSpec  ExternalSaturationOutDataTypeStr=Inherit: Same as second input  DerivativeSourceVariant=Disabled  PreIntVariant=InternalPreInt
  PID Controller5 : slpidlib/PID Controller  Controller=PI  Form=Parallel  TimeDomain=Discrete-time  UseExternalTs=off  SampleTime=SampleTime  IntegratorMethod=Forward Euler  FilterMethod=Forward Euler  ControllerParametersSource=internal  P=10  I=20  UseKiTs=off  D=0  UseExternalDerivativeSource=off  N=100  UseFilter=on  TunerSelectOption=Transfer Function Based (PID Tuner App)  InitialConditionSource=internal  InitialConditionForIntegrator=0  InitialConditionForFilter=0  DifferentiatorICPrevScaledInput=0  ExternalReset=none  TrackingMode=off  Kt=1  LimitOutput=off  SatLimitsSource=internal  UpperSaturationLimit=inf  LowerSaturationLimit=-inf  LinearizeAsGain=on  AntiWindupMode=none  Kb=1  LimitIntegrator=off  UpperIntegratorSaturationLimit=inf  LowerIntegratorSaturationLimit=-inf  POutMin=[]  POutMax=[]  IOutMin=[]  IOutMax=[]  DOutMin=[]  DOutMax=[]  NOutMin=[]  NOutMax=[]  SumOutMin=[]  SumOutMax=[]  SaturationOutMin=[]  SaturationOutMax=[]  PParamMin=[]  PParamMax=[]  IParamMin=[]  IParamMax=[]  DParamMin=[]  DParamMax=[]  NParamMin=[]  NParamMax=[]  KbParamMin=[]  KbParamMax=[]  KtParamMin=[]  KtParamMax=[]  KbOutMin=[]  KbOutMax=[]  KtOutMin=[]  KtOutMax=[]  IntegratorOutMin=[]  IntegratorOutMax=[]  FilterOutMin=[]  FilterOutMax=[]  SumI1OutMin=[]  SumI1OutMax=[]  SumI2OutMin=[]  SumI2OutMax=[]  SumI3OutMin=[]  SumI3OutMax=[]  SumI4OutMin=[]  SumI4OutMax=[]  SumDOutMin=[]  SumDOutMax=[]  DifferentiatorOutMin=[]  DifferentiatorOutMax=[]  FilterDiffOutCoefMin=[]  FilterDiffOutCoefMax=[]  ReciprocalOutMin=[]  ReciprocalOutMax=[]  SumDenOutMin=[]  SumDenOutMax=[]  SumNumOutMin=[]  SumNumOutMax=[]  DivideOutMin=[]  DivideOutMax=[]  UdiffTsProdOutMin=[]  UdiffTsProdOutMax=[]  NTsProdOutMin=[]  NTsProdOutMax=[]  UintegralTsProdOutMin=[]  UintegralTsProdOutMax=[]  UngainTsProdOutMin=[]  UngainTsProdOutMax=[]  ClampingZeroOutDataTypeStr=Inherit: Inherit via back propagation  ClampingZeroOutMin=[]  ClampingZeroOutMax=[]  FilterDenConstantOutDataTypeStr=Inherit: Inherit via back propagation  FilterDenConstantOutMin=[]  FilterDenConstantOutMax=[]  PCopyOutDataTypeStr=Inherit: Inherit via back propagation  PCopyOutMin=[]  PCopyOutMax=[]  NCopyOutDataTypeStr=Inherit: Inherit via back propagation  NCopyOutMin=[]  NCopyOutMax=[]  IntegratorContinuousStateAttributes=''  IntegratorStateMustResolveToSignalObject=off  IntegratorRTWStateStorageClass=Auto  FilterContinuousStateAttributes=''  FilterStateMustResolveToSignalObject=off  FilterRTWStateStorageClass=Auto  ParallelPVariant=InternalParameters  IdealPVariant=Disabled  IVariant=InternalParameters  DVariant=Disabled  IntegratorVariant=Discrete  SatVariant=Disabled  AWVariant=Passthrough  PCopyVariant=Disabled  TRVariant=Disabled  FdbkBlocksVariant=Forward  IdealPFdbkVariant=Disabled  SatFdbkVariant=Disabled  DerivativeFilterVariant=Disabled  NVariant=Disabled  NCopyVariant=Disabled_SignalSpec  FilterICVariant=Disabled  IntegratorICVariant=InternalICs  ExternalResetVariant=Disabled  TRSumVariant=Passthrough  SumFdbkVariant=Disabled  SumVariant=Sum_PI  TsampFilterVariant=InternalTs  TsampNgainVariant=Passthrough  TsampIntegralVariant=Disabled_SignalSpec  ExternalSaturationOutDataTypeStr=Inherit: Same as second input  DerivativeSourceVariant=Disabled  PreIntVariant=InternalPreInt
  PSS model : Constant  SampleTime=SampleTime
  "PV ( V, I, P )" : Scope  NumInputPorts=3
  "PV ( V, I, P )1" : Scope
  "PV ( V, I, P )2" : Scope  NumInputPorts=3
  "PV ( V, I, P )3" : Scope  NumInputPorts=2
  "PV ( V, I, P )4" : Scope
  PV Array1 : Subsystem  LoadFcn=sps_rtmsupport('LoadFcn',gcbh);  StartFcn=sps_rtmsupport('StartFcn',gcbh);  StopFcn=sps_rtmsupport('StopFcn',gcbh);  mask(PV array){Npar=3500, Nser=11, PlotType=array @ 1000 W/m2 & specified temperatures, S_vec=[ 1000  500  100 ], Temp_C_vec=[ 45 25  ], ModuleName=REC Solar REC215PE (BLK), PlotWhenSelected=off, Pm=215.08, Ncell=60, Voc=36.3, Isc=8.1, Vm=28.3, Im=7.6, beta_Voc_pc=-0.318, alpha_Isc_pc=0.011, beta_Voc=-0.11543, alpha_Isc=0.000891, IL=8.1095, I0=5.3883e-11, nI=0.9153, Rsh=438.7897, Rs=0.51188, RobustModel=off, RobustCellTemperature=313.3991, BAL=on, Tc=1e-6, Tfilter=5e-5}
      mask prompts: Npar "Parallel strings"; Nser "Series-connected modules per string"; S_vec "Irradiances (W/m2)"; Temp_C_vec "T_cell (deg. C)"; ModuleName "Module:"; PlotWhenSelected "Plot I-V and P-V characteristics when a module is selected"; Pm "Maximum Power (W)"; Ncell "Cells per module (Ncell)"; Voc "Open circuit voltage  Voc (V)"; Isc "Short-circuit current Isc (A)"; Vm "Voltage at maximum power point Vmp (V)"; Im "Current at maximum power point Imp (A)"; beta_Voc_pc "Temperature coefficient of Voc (%/deg.C)"; alpha_Isc_pc "Temperature coefficient of Isc (%/deg.C)"; beta_Voc "Temperature coefficient of Voc (V/deg.C)"; alpha_Isc "Temperature coefficient of Isc (A/deg.C)"; IL "Light-generated current IL (A)"; I0 "Diode saturation current I0 (A)"; nI "Diode ideality factor"; Rsh "Shunt resistance Rsh (ohms)"; Rs "Series resistance Rs (ohms)"; RobustModel "Robust discrete model"; RobustCellTemperature "Cell temperature, in deg.C. (input 2 is disabled)"; BAL "Break algebraic loop in internal model"; Tc "Break loop time constant (s)"; Tfilter "Measurement filter time constant (s)"
      mask help:
      | Implements a PV array built of strings of PV modules connected in parallel. Each string consists of modules connected in series.
      | Allows modeling of a variety of preset PV modules available from NREL System Advisor Model (Jan. 2014) as well as user-defined PV module.
      |
      | Input 1 = Sun irradiance, in W/m2, and input 2 = Cell temperature, in deg.C.
      mask init:
      | Block = gcb;
      | [k,k1,q,Tref_C,Tref_K,EgRef,dEgdT,Rsh_array5pc,VT_ref,Tsf,Tf,VIdiodePV,WantBlockChoice] = PVArrayInit(Block, Nser, Npar, Ncell, Rsh, nI, Tfilter, Voc, I0);
      | powericon('SetInternalModels','set',Block,WantBlockChoice);
      | sps_rtmsupport('parametereditingmodes',Block, [3 6 7 23]);
      settings: CopyFcn=sps_rtmsupport('CopyFcn',gcbh);  DeleteFcn=sps_rtmsupport('DeleteFcn',gcbh);  UndoDeleteFcn=sps_rtmsupport('UndoDeleteFcn',gcbh);  ModelCloseFcn=sps_rtmsupport('ModelCloseFcn',gcbh);  PreSaveFcn=sps_rtmsupport('PreSaveFcn',gcbh);  PostSaveFcn=sps_rtmsupport('PostSaveFcn',gcbh);  NameChangeFcn=sps_rtmsupport('NameChangeFcn',gcbh);  PreCopyFcn=sps_rtmsupport('PreCopyFcn',gcbh);  CloseFcn=sps_rtmsupport('CloseFcn',gcbh);  PreDeleteFcn=sps_rtmsupport('PreDeleteFcn',gcbh);
      settings: OpenFcn=|
      | %assignin('base','PVMaskOpening',1);
      | %open_system(gcb,'mask')
      | %assignin('base','PVMaskOpening',0);
      | sps_rtmsupport('OpenFcn',gcbh, [3 6 7 23]);
      mask Help: helpview(psbhelp);
      mask TypeOptions PlotType: one module @ 25 deg.C & specified irradiances | array @ 25 deg.C & specified irradiances | array @ 1000 W/m2 & specified temperatures
      mask Callback PlotType: PVArrayCback(gcb)
